simulink model "FBL_commonP_circle"  (R2025a)
settings: Solver=VariableStepAuto  StartTime=0.0  StopTime=240  RelTol=1e-3
undefined symbols (not defined in the file or in its folder): National_Instruments, PCI
libraries: sldrtlib x3, simulink x1
settings Model: Creator=dperera  LastModifiedBy=dperera

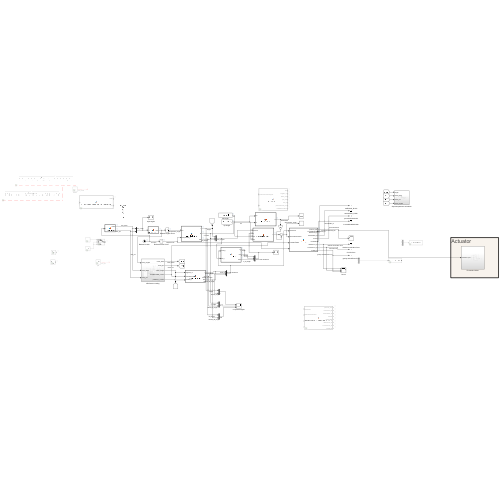
[thumbnail: Simulink's stored preview of the top-level diagram]
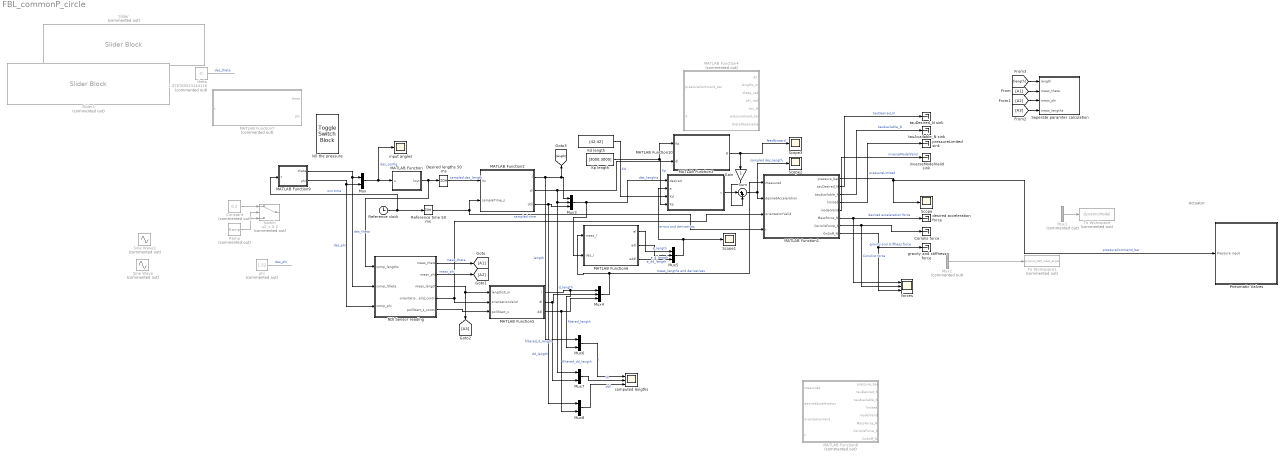
== system FBL_commonP_circle ==
  note: Actuator
  Constant : Constant  Commented=on  Value=0.2
  Coriolis force : Terminator
  Desired lengths 50 ms : ZeroOrderHold  SampleTime=0.05
  Gain : Gain
  Kd length : Constant  Value=[42;42]
  Kp length : Constant  Value=[3000;3000]
  MATLAB Function : MATLAB Function  TreatAsAtomicUnit=on
  MATLAB Function1 : MATLAB Function  TreatAsAtomicUnit=on
  MATLAB Function10 : MATLAB Function  TreatAsAtomicUnit=on
  MATLAB Function2 : MATLAB Function  TreatAsAtomicUnit=on
  MATLAB Function3 : MATLAB Function  TreatAsAtomicUnit=on
  MATLAB Function4 : MATLAB Function  Commented=on  TreatAsAtomicUnit=on
  MATLAB Function5 : MATLAB Function  TreatAsAtomicUnit=on
  MATLAB Function6 : MATLAB Function  TreatAsAtomicUnit=on
  MATLAB Function7 : MATLAB Function  Commented=on  TreatAsAtomicUnit=on
  MATLAB Function8 : MATLAB Function  Commented=on  TreatAsAtomicUnit=on
  MATLAB Function9 : MATLAB Function  TreatAsAtomicUnit=on
  Mux{,6..8} (4 alike) : Mux  Inputs=2
  Mux1 : Mux  Commented=on
  Mux2 : Mux  Commented=on
  Mux3 : Mux  Inputs=3
  Mux4 : Mux  Inputs=3
  Mux5 : Mux  Inputs=3
  NDI Sensor reading : Subsystem
  Pneumatic Valves : Subsystem
  Ramp : simulink/Sources/Ramp  Commented=on  slope=0.2/5  start=1  InitialOutput=0
  Reference clock : Clock
  Reference time 50 ms : ZeroOrderHold  SampleTime=0.05
  Scope{,1..3} (4 alike) : Scope
      Scope settings: ActiveDisplayYMinimum=-0.37334273695648185  ActiveDisplayYMaximum=3.3600846326083369  DataLoggingVariableName=ScopeData6
      Scope1 settings: ActiveDisplayYMinimum=-0.019338012914829127  ActiveDisplayYMaximum=0.016644783463870338  DataLoggingVariableName=ScopeData8
      Scope2 settings: ActiveDisplayYMinimum=-1  ActiveDisplayYMaximum=1  DataLoggingVariableName=ScopeData9
      Scope3 settings: ActiveDisplayYMinimum=-5.4117919345695178  ActiveDisplayYMaximum=5.4108217557534957  DataLoggingVariableName=ScopeData13
  Seperate paramter calculation : Subsystem
  Sine Wave : Sin  Commented=on  Amplitude=1.5  Bias=1.5  Frequency=0.2  Phase=3*pi/2  SampleTime=0
  Sine Wave1 : Sin  Commented=on  Amplitude=1.5  Bias=1.5  Frequency=0.2  Phase=3*pi/2  SampleTime=0
  Slider : SliderBlock  Commented=on  ScaleMin=-3.14  ScaleMax=3.14
  Slider1 : SliderBlock  Commented=on  ScaleMax=3.14
  Sum : Sum  Inputs=|++
  Switch : Switch  Commented=on  Criteria=u2 > Threshold  Threshold=0.2  SaturateOnIntegerOverflow=off  InputSameDT=off
  To Workspace : ToWorkspace  Commented=on  VariableName=dynamicModel  SaveFormat=Timeseries  SampleTime=-1
  To Workspace1 : ToWorkspace  Commented=on  VariableName=dynamic_NDI_meas_angle  SaveFormat=Timeseries  SampleTime=-1
  computed lengths : Scope  NumInputPorts=3
      settings: ActiveDisplayYMinimum=-0.0163263543588523  ActiveDisplayYMaximum=0.016938688313851029  DataLoggingVariableName=ScopeData11
  desired acceleration force : Terminator
  forces : Scope  NumInputPorts=3
      settings: ActiveDisplayYMinimum=-26.920603597626503  ActiveDisplayYMaximum=23.728678964344354  DataLoggingVariableName=ScopeData10
  gravity and stiffness force : Terminator
  input angles : Scope
      settings: ActiveDisplayYMinimum=-0.19634954084936201  ActiveDisplayYMaximum=1.7671458676442586  DataLoggingVariableName=ScopeData12
  inverseModelValid sink : Terminator
  kill the pressure : ToggleSwitchBlock
  phi : Constant  Commented=on  Value=1.52
  pressureLimited sink : Terminator
  tauAvailable_N sink : Terminator
  tauDesired_N sink : Terminator
  theta : Constant  Commented=on  Value=1.076760523144116
  wires:
  Mux/1 -> input angles/1, MATLAB Function/1(u)  "des_config"
  MATLAB Function9/1(theta) -> NDI Sensor reading/2(comp_ltheta), Mux/1  "des_theta"
  Mux1/1 -> To Workspace/1
  Mux2/1 -> To Workspace1/1
  MATLAB Function/1(lout) -> Desired lengths 50 ms/1, NDI Sensor reading/1(comp_lengths)
  NDI Sensor reading/3(meas_length) -> MATLAB Function5/1(lengths3_m), [A3]
  MATLAB Function2/1(l) -> Mux6/1, Mux3/1, [length]  "length"
  MATLAB Function2/2(dl) -> MATLAB Function10/2(dl), Mux7/1, Mux3/2  "d_length"
  MATLAB Function2/3(ddl) -> Mux8/1, Mux3/3  "dd_length"
  MATLAB Function5/1(l) -> Mux6/2, Mux4/1  "fitered_length"
  MATLAB Function5/2(dl) -> Mux7/2, Mux4/2  "filtered_d_length"
  MATLAB Function5/3(ddl) -> Mux8/2, Mux4/3  "filtered_dd_length"
  Mux4/1 -> MATLAB Function1/1(measured), MATLAB Function6/1(meas_l)  "meas_lengths and derivatives"
  Mux3/1 -> MATLAB Function3/1(desired), MATLAB Function6/2(des_l)  "des_lenghts"
  MATLAB Function6/2(edl) -> Mux5/2  "e_d_length"
  MATLAB Function6/1(el) -> Mux5/1  "e_length"
  MATLAB Function6/3(eddl) -> Mux5/3  "e_dd_length"
  Mux5/1 -> MATLAB Function3/2(e), Scope1/1  "errors and derivatives"
  Desired lengths 50 ms/1 -> MATLAB Function2/1(lIn)  "sampled des_length"
  Reference clock/1 -> MATLAB Function9/1(t), Reference time 50 ms/1  "sim time"
  Reference time 50 ms/1 -> MATLAB Function1/4(t), MATLAB Function2/2(sampleTime_s)  "sampled time"
  NDI Sensor reading/4(orientationValid_control) -> MATLAB Function1/3(orientationValid), MATLAB Function5/2(orientationValid)
  NDI Sensor reading/5(pollStart_s_control) -> MATLAB Function5/3(pollStart_s)
  Kd length/1 -> MATLAB Function3/3(Kd)  "Kd"
  Kp length/1 -> MATLAB Function10/1(Kp), MATLAB Function3/4(Kp)  "Kp"
  MATLAB Function3/1(v) -> Sum/1
  MATLAB Function1/1(pressure_bar) -> Scope/1, Pneumatic Valves/1(Pressure input)  "pressureCommand_bar"
  MATLAB Function1/2(tauDesired_N) -> tauDesired_N sink/1  "tauDesired_N"
  MATLAB Function1/3(tauAvailable_N) -> tauAvailable_N sink/1  "tauAvailable_N"
  MATLAB Function1/4(limited) -> pressureLimited sink/1  "pressureLimited"
  MATLAB Function1/5(modelValid) -> inverseModelValid sink/1  "inverseModelValid"
  NDI Sensor reading/1(meas_theta) -> [A1]  "meas_theta"
  [A1] -> Seperate paramter calculation/2(meas_theta)
  NDI Sensor reading/2(meas_phi) -> [A2]  "meas_phi"
  [A2] -> Seperate paramter calculation/3(meas_phi)
  [A3] -> Seperate paramter calculation/4(meas_lengths)
  [length] -> Seperate paramter calculation/1(length)
  MATLAB Function1/6(MassForce_N) -> forces/1, desired acceleration force/1  "desired acceleration force"
  MATLAB Function1/7(CoriolisForce_N) -> forces/2, Coriolis force/1  "Coriolist force"
  MATLAB Function1/8(GnStiff_N) -> forces/3, gravity and stiffness force/1  "gravity and stiffness force"
  Mux6/1 -> computed lengths/1  "l"
  Mux7/1 -> computed lengths/2  "dl"
  Mux8/1 -> computed lengths/3  "ddl"
  Ramp/1 -> Switch/2, Switch/3
  Constant/1 -> Switch/1
  theta/1 -> ?  "des_theta"
  phi/1 -> ?  "des_phi"
  MATLAB Function9/2(phi) -> NDI Sensor reading/3(comp_phi), Mux/2  "des_phi"
  MATLAB Function10/1(ff) -> Scope3/1, Gain/1  "feedforward"
  Sum/1 -> MATLAB Function1/2(desiredAcceleration), Scope2/1  "sampled des_length"
  Gain/1 -> Sum/2

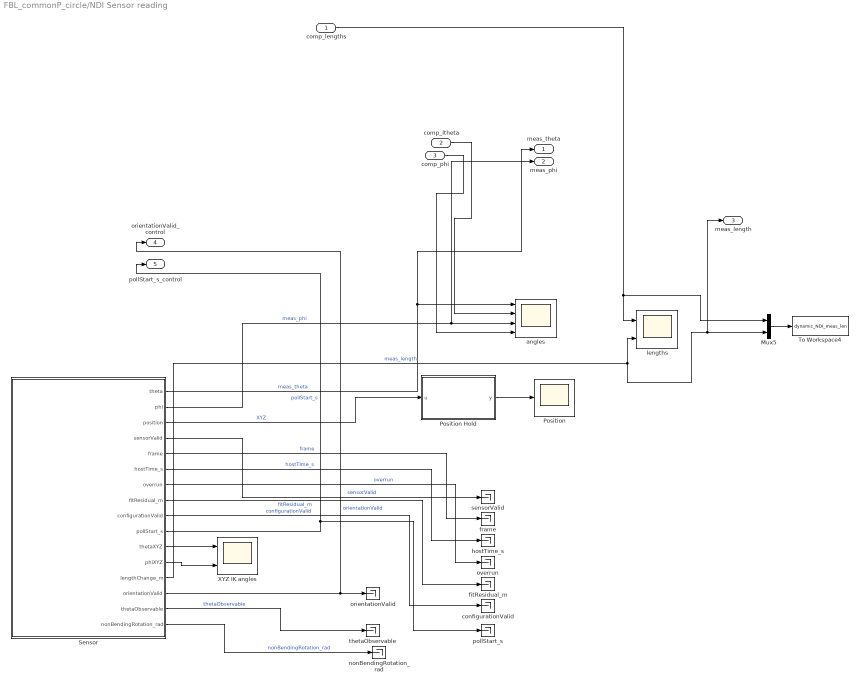
== system FBL_commonP_circle/NDI Sensor reading ==
  comp_lengths : Inport
  comp_ltheta : Inport  Port=2
  comp_phi : Inport  Port=3
  Mux5 : Mux  Inputs=2
  Position : Scope
      settings: ActiveDisplayYMinimum=-0.21656345474719998  ActiveDisplayYMaximum=0.33777835857868188
  Position Hold : MATLAB Function  TreatAsAtomicUnit=on
  Sensor : Subsystem
  To Workspace4 : ToWorkspace  VariableName=dynamic_NDI_meas_len  SaveFormat=Timeseries  SampleTime=-1
  XYZ IK angles : Scope  NumInputPorts=2
      settings: DataLoggingVariableName=ScopeData2
  angles : Scope  NumInputPorts=4
      settings: ActiveDisplayYMinimum=-3.523325206652153  ActiveDisplayYMaximum=4.312344616749975
  configurationValid : Terminator
  fitResidual_m : Terminator
  frame : Terminator
  hostTime_s : Terminator
  lengths : Scope  NumInputPorts=2
      settings: ActiveDisplayYMinimum=-0.0017146774565175815  ActiveDisplayYMaximum=0.0020057370608089205  DataLoggingVariableName=ScopeData3
  nonBendingRotation_rad : Terminator
  orientationValid : Terminator
  overrun : Terminator
  pollStart_s : Terminator
  sensorValid : Terminator
  thetaObservable : Terminator
  meas_theta : Outport
  meas_phi : Outport  Port=2
  meas_length : Outport  Port=3
  orientationValid_control : Outport  Port=4
  pollStart_s_control : Outport  Port=5
  wires:
  Sensor/13(lengthChange_m) -> lengths/2, meas_length/1, Mux5/2  "meas_length"
  comp_lengths/1 -> lengths/1, Mux5/1
  Sensor/10(pollStart_s) -> pollStart_s/1, pollStart_s_control/1  "pollStart_s"
  Sensor/2(phi) -> angles/3, meas_phi/1  "meas_phi"
  Sensor/3(position) -> Position Hold/1(u)  "XYZ"
  Sensor/1(theta) -> meas_theta/1, angles/1  "meas_theta"
  Sensor/6(hostTime_s) -> hostTime_s/1  "hostTIme_s"
  Sensor/9(configurationValid) -> configurationValid/1  "configurationValid"
  Sensor/4(sensorValid) -> sensorValid/1  "sensorValid"
  Sensor/7(overrun) -> overrun/1  "overrun"
  Sensor/5(frame) -> frame/1  "frame"
  comp_ltheta/1 -> angles/2
  Sensor/8(fitResidual_m) -> fitResidual_m/1  "fitResidual_m"
  Sensor/12(phiXYZ) -> XYZ IK angles/2
  Sensor/11(thetaXYZ) -> XYZ IK angles/1
  Position Hold/1(y) -> Position/1
  Mux5/1 -> To Workspace4/1
  Sensor/14(orientationValid) -> orientationValid_control/1, orientationValid/1  "orientationValid"
  Sensor/16(nonBendingRotation_rad) -> nonBendingRotation_rad/1  "nonBendingRotation_rad"
  Sensor/15(thetaObservable) -> thetaObservable/1  "thetaObservable"
  comp_phi/1 -> angles/4

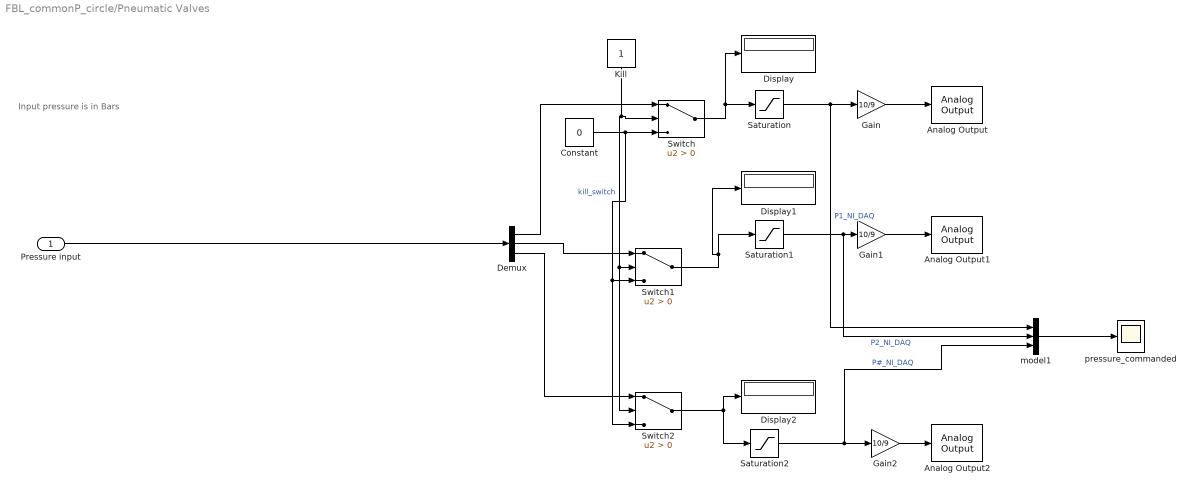
== system FBL_commonP_circle/Pneumatic Valves ==
  note: Input pressure is in Bars
  Pressure input : Inport
  Analog Output : sldrtlib/Analog Output  SampleTime=1/100  MaxMissedTicks=inf  ShowMissedTicks=off  YieldWhenWaiting=off  DrvName=National_Instruments/PCI-6703  DrvAddress=4294967295  DrvOptions=0  Channels=1  RangeMode=1  VoltRange=1  InitialValue=0  FinalValue=0
      settings: AttributesFormatString=National Instruments\nPCI-6703 [auto]
  Analog Output1 : sldrtlib/Analog Output  SampleTime=1/100  MaxMissedTicks=inf  ShowMissedTicks=off  YieldWhenWaiting=off  DrvName=National_Instruments/PCI-6703  DrvAddress=4294967295  DrvOptions=0  Channels=2  RangeMode=1  VoltRange=1  InitialValue=0  FinalValue=0
      settings: AttributesFormatString=National Instruments\nPCI-6703 [auto]
  Analog Output2 : sldrtlib/Analog Output  SampleTime=1/100  MaxMissedTicks=inf  ShowMissedTicks=off  YieldWhenWaiting=off  DrvName=National_Instruments/PCI-6703  DrvAddress=4294967295  DrvOptions=0  Channels=3  RangeMode=1  VoltRange=1  InitialValue=0  FinalValue=0
      settings: AttributesFormatString=National Instruments\nPCI-6703 [auto]
  Constant : Constant  Value=0
  Demux : Demux  Outputs=3
  Display : Display
  Display1 : Display
  Display2 : Display
  Gain : Gain  Gain=10/9
  Gain1 : Gain  Gain=10/9
  Gain2 : Gain  Gain=10/9
  Kill : Constant
  Saturation : Saturate  UpperLimit=3  LowerLimit=0
  Saturation1 : Saturate  UpperLimit=3  LowerLimit=0
  Saturation2 : Saturate  UpperLimit=3  LowerLimit=0
  Switch : Switch  Criteria=u2 > Threshold  SaturateOnIntegerOverflow=off  InputSameDT=off
  Switch1 : Switch  Criteria=u2 > Threshold  SaturateOnIntegerOverflow=off  InputSameDT=off
  Switch2 : Switch  Criteria=u2 > Threshold  SaturateOnIntegerOverflow=off  InputSameDT=off
  model1 : Mux  Inputs=3
  pressure_commanded : Scope
      settings: ActiveDisplayYMinimum=-0.37499999999999989  ActiveDisplayYMaximum=3.375  DataLoggingVariableName=ScopeData7
  wires:
  Constant/1 -> Switch2/3, Switch1/3, Switch/3
  Kill/1 -> Switch2/2, Switch1/2, Switch/2  "kill_switch"
  Switch/1 -> Display/1, Saturation/1
  Gain/1 -> Analog Output/1
  Saturation/1 -> model1/1, Gain/1  "P1_NI_DAQ"
  Demux/3 -> Switch2/1
  Gain1/1 -> Analog Output1/1
  Gain2/1 -> Analog Output2/1
  Saturation2/1 -> model1/3, Gain2/1  "P#_NI_DAQ"
  Switch2/1 -> Saturation2/1, Display2/1
  Demux/2 -> Switch1/1
  Switch1/1 -> Saturation1/1, Display1/1
  model1/1 -> pressure_commanded/1
  Saturation1/1 -> model1/2, Gain1/1  "P2_NI_DAQ"
  Demux/1 -> Switch/1
  Pressure input/1 -> Demux/1

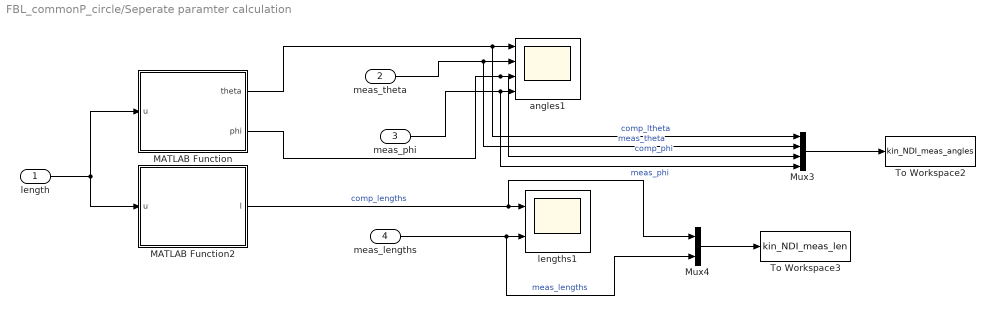
== system FBL_commonP_circle/Seperate paramter calculation ==
  length : Inport
  meas_theta : Inport  Port=2
  meas_phi : Inport  Port=3
  meas_lengths : Inport  Port=4
  MATLAB Function : MATLAB Function  TreatAsAtomicUnit=on
  MATLAB Function2 : MATLAB Function  TreatAsAtomicUnit=on
  Mux3 : Mux
  Mux4 : Mux  Inputs=2
  To Workspace2 : ToWorkspace  VariableName=kin_NDI_meas_angles  SaveFormat=Timeseries  SampleTime=-1
  To Workspace3 : ToWorkspace  VariableName=kin_NDI_meas_len  SaveFormat=Timeseries  SampleTime=-1
  angles1 : Scope  NumInputPorts=4
      settings: ActiveDisplayYMinimum=-3.9269137322662839  ActiveDisplayYMaximum=3.9265599408279468  DataLoggingVariableName=ScopeData4
  lengths1 : Scope  NumInputPorts=2
      settings: ActiveDisplayYMinimum=-0.02243223759551808  ActiveDisplayYMaximum=0.037530111947788623  DataLoggingVariableName=ScopeData5
  wires:
  meas_lengths/1 -> Mux4/2, lengths1/2  "meas_lengths"
  meas_theta/1 -> Mux3/2, angles1/2  "meas_theta"
  MATLAB Function/2(phi) -> Mux3/3, angles1/3  "comp_phi"
  Mux3/1 -> To Workspace2/1
  meas_phi/1 -> Mux3/4, angles1/4  "meas_phi"
  MATLAB Function/1(theta) -> Mux3/1, angles1/1  "comp_ltheta"
  Mux4/1 -> To Workspace3/1
  MATLAB Function2/1(l) -> Mux4/1, lengths1/1  "comp_lengths"
  length/1 -> MATLAB Function2/1(u), MATLAB Function/1(u)

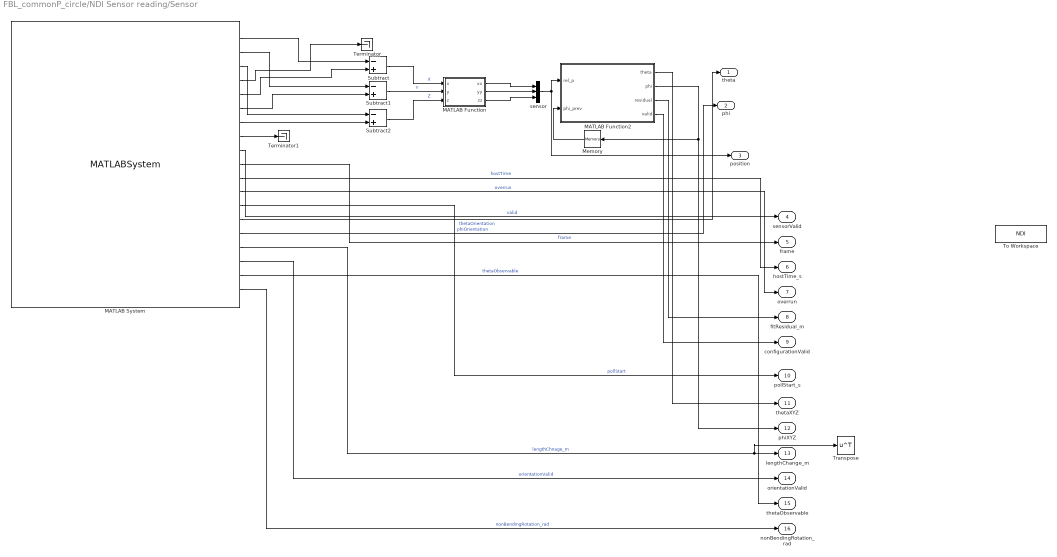
== system FBL_commonP_circle/NDI Sensor reading/Sensor ==
  MATLAB Function : MATLAB Function  TreatAsAtomicUnit=on
  MATLAB Function2 : MATLAB Function  TreatAsAtomicUnit=on
  MATLAB System : MATLABSystem  System=AuroraReader_s2_Position_only  Port=COM12  BaudRate=ndiConfig.BaudRate  SamplePeriod=ndiConfig.SamplePeriod  BaseSensorId=0A  TipSensorId=0B  CalibrationFile=C:\Users\dperera\OneDrive - Texas A&M University\Lab\Research\fDyn_ExpCom\hyDyn_Ctrl\ndi_orientation_recordings\calibration_20260930_190505_898.mat  PreflightSeconds=5  ActuatorRadius=0.013  SimulateUsing=Interpreted execution
      mask Type: AuroraReader_s2_Position_only
  Memory : Memory  InitialCondition=0.0001
  Subtract : Sum  Inputs=-+
  Subtract1 : Sum  Inputs=-+
  Subtract2 : Sum  Inputs=-+
  Terminator : Terminator
  Terminator1 : Terminator
  To Workspace : ToWorkspace  VariableName=NDI  SaveFormat=Timeseries  SampleTime=-1
  Transpose : Math  Operator=transpose
  sensor : Mux  Inputs=3
  theta : Outport
  phi : Outport  Port=2
  position : Outport  Port=3
  sensorValid : Outport  Port=4
  frame : Outport  Port=5
  hostTime_s : Outport  Port=6
  overrun : Outport  Port=7
  fitResidual_m : Outport  Port=8
  configurationValid : Outport  Port=9
  pollStart_s : Outport  Port=10
  thetaXYZ : Outport  Port=11
  phiXYZ : Outport  Port=12
  lengthChange_m : Outport  Port=13
  orientationValid : Outport  Port=14
  thetaObservable : Outport  Port=15
  nonBendingRotation_rad : Outport  Port=16
  wires:
  MATLAB System/2 -> Subtract1/1
  MATLAB Function/3(zz) -> sensor/3
  Subtract1/1 -> MATLAB Function/2(y)  "Y"
  Subtract2/1 -> MATLAB Function/3(z)  "Z"
  MATLAB System/5 -> Subtract/2
  sensor/1 -> position/1, MATLAB Function2/1(rel_p)
  MATLAB System/8 -> Terminator1/1
  MATLAB Function/1(xx) -> sensor/1
  Subtract/1 -> MATLAB Function/1(x)  "X"
  MATLAB Function/2(yy) -> sensor/2
  MATLAB System/1 -> Subtract/1
  MATLAB Function2/2(phi) -> Memory/1, phiXYZ/1
  MATLAB System/7 -> Subtract2/2
  MATLAB System/4 -> Terminator/1
  MATLAB System/3 -> Subtract2/1
  MATLAB System/6 -> Subtract1/2
  Memory/1 -> MATLAB Function2/2(phi_prev)
  MATLAB System/9 -> sensorValid/1  "valid"
  MATLAB System/11 -> hostTime_s/1  "hostTime"
  MATLAB System/12 -> overrun/1  "overrun"
  MATLAB Function2/3(residual) -> fitResidual_m/1
  MATLAB Function2/4(valid) -> configurationValid/1
  MATLAB System/13 -> pollStart_s/1  "pollStart"
  MATLAB System/14 -> theta/1  "thetaOrientation"
  MATLAB System/15 -> phi/1  "phiOrientation"
  MATLAB Function2/1(theta) -> thetaXYZ/1
  MATLAB System/16 -> Transpose/1, lengthChange_m/1  "lengthChnage_m"
  MATLAB System/17 -> orientationValid/1  "orientationValid"
  MATLAB System/18 -> thetaObservable/1  "thetaObservable"
  MATLAB System/19 -> nonBendingRotation_rad/1  "nonBendingRotation_rad"
  MATLAB System/10 -> frame/1  "frame"

== matlab function FBL_commonP_circle/MATLAB Function2 ==
  data: lIn input; l output; dl output; ddl output; sampleTime_s input
function [l, dl, ddl] = lengthDerivatives(lIn, sampleTime_s)
%#codegen
% Desired reduced lengths [l2;l3] in m; derivatives in m/s and m/s^2.
% sampleTime_s is a 0.05 s zero-order-held Clock signal.
persistent lastL lastT velocity acceleration
if isempty(lastT)
    lastL = zeros(2,1);
    lastT = -1;
    velocity = zeros(2,1);
    acceleration = zeros(2,1);
end
l = lastL;
dl = velocity;
ddl = acceleration;
if ~all(isfinite(lIn)) || ~isfinite(sampleTime_s)
    return;
end
q = [lIn(1); lIn(2)];
if lastT < 0
    lastL = q;
    lastT = sampleTime_s;
    l = q;
    return;
end
dt = sampleTime_s - lastT;
if dt > 1e-6
    rawVelocity = (q-lastL)/dt;
    oldVelocity = velocity;
    alphaV = dt/(0.10+dt);
    velocity = velocity + alphaV*(rawVelocity-velocity);
    rawAcceleration = (velocity-oldVelocity)/dt;
    alphaA = dt/(0.15+dt);
    acceleration = acceleration + alphaA*(rawAcceleration-acceleration);
    lastL = q;
    lastT = sampleTime_s;
end
l = lastL;
dl = velocity;
ddl = acceleration;
end

== matlab function FBL_commonP_circle/MATLAB Function3 ==
  data: desired input; v output; e input; Kd input; Kp input
function v = feedbacklinearization(desired, e, Kd, Kp)
%#codegen
% v = desired acceleration + Kd*velocity error + Kp*position error.
% desired,e: [l2;l3;dl2;dl3;ddl2;ddl3]; gains are 2-vectors.
% Kd units 1/s, Kp units 1/s^2; v units m/s^2.
v = zeros(2,1);
if ~all(isfinite(desired)) || ~all(isfinite(e)) || ...
        ~all(isfinite(Kd)) || ~all(isfinite(Kp)) || ...
        any(Kd < 0) || any(Kp < 0)
    return;
end
v = desired(5:6) + Kd(:).*e(3:4) + Kp(:).*e(1:2);
end

== matlab function FBL_commonP_circle/MATLAB Function4 ==
  data: pressureCommand_bar input; X input; dX output; lengths_m output; theta_rad output; phi_rad output; tau_N output; pressureUsed_bar output; thetaObservable output
% function dX  = DynamicModel(p, X)
%#codegen
% This file computes length velocity and accelration from pressures using the dynamic model.
%
% Inputs:
%   p   : pressures [3x1] (Pa)
%   X   : length derivatives [4x1] (m)
%         [l2; l3; dl2; dl3]
%
% Output:
%   dX  : length derivatives [4x1] (m)
%         [dl2; dl3; ddl2; ddl3]

function [dX, lengths_m, theta_rad, phi_rad, tau_N, ...
          pressureUsed_bar, thetaObservable] = forwardModel(pressureCommand_bar, X)
%#codegen
% pressureCommand_bar = [P1; P2; P3], nonnegative bar
% X = [l2; l3; dl2; dl3], with l1 = -l2-l3

L = 0.17411;
r = 0.013; % PMA radial offset from backbone (m)
mass = 0.1;
K = 1350 * [2 1; 1 2];
D = 40 * eye(2);
gArm = [0; 0; -9.81];
mu = 2000;
lengthBounds = [-0.035; 0.035; 1e6];

pressureUsed_bar = min(max(pressureCommand_bar, 0), 3);
pressureDiameter_m = 0.013; % Effective pressure-area diameter, independent of r
pressureRadius_m = pressureDiameter_m/2;
area = pi * pressureRadius_m^2;

% Positive P1, P2, P3 give the established -X, -60°, +60°
% nominal bending directions, respectively.
tau_N = area * 1e5 * [-1 1 0; -1 0 1] * pressureUsed_bar;

dX = armS_single_entry(0, X, L, r, mass, gArm, ...
                       K, D, tau_N, mu, lengthBounds);

l2 = X(1);
l3 = X(2);
lengths_m = [-l2-l3; l2; l3];

u = (l2+l3)/r;
v = (l3-l2)/(sqrt(3)*r);
phi_rad = hypot(u, v);
theta_rad = atan2(v, u);
thetaObservable = phi_rad > 0.5*pi/180;


end

== matlab function FBL_commonP_circle/MATLAB Function5 ==
  data: lengths3_m input; l output; dl output; ddl output; orientationValid input; pollStart_s input
function [l, dl, ddl] = filteredDerivatives(lengths3_m, orientationValid, pollStart_s)
%#codegen
% NDI lengths are [l1;l2;l3]; model coordinates are [l2;l3].
% Invalid or repeated BX frames do not update the derivative states.
persistent lastL lastT velocity acceleration
if isempty(lastT)
    lastL = nan(2,1);
    lastT = -1;
    velocity = zeros(2,1);
    acceleration = zeros(2,1);
end
l = lastL;
dl = velocity;
ddl = acceleration;
if ~orientationValid || ~all(isfinite(lengths3_m)) || ~isfinite(pollStart_s)
    return;
end
q = [lengths3_m(2); lengths3_m(3)];
if lastT < 0
    lastL = q;
    lastT = pollStart_s;
    l = q;
    return;
end
dt = pollStart_s-lastT;
if dt > 1e-6
    rawVelocity = (q-lastL)/dt;
    oldVelocity = velocity;
    alphaV = dt/(0.20+dt);
    velocity = velocity + alphaV*(rawVelocity-velocity);
    rawAcceleration = (velocity-oldVelocity)/dt;
    alphaA = dt/(0.30+dt);
    acceleration = acceleration + alphaA*(rawAcceleration-acceleration);
    lastL = q;
    lastT = pollStart_s;
end
l = lastL;
dl = velocity;
ddl = acceleration;
end

== matlab function FBL_commonP_circle/MATLAB Function6 ==
  data: meas_l input; el output; edl output; eddl output; des_l input
function [el, edl, eddl] = computeLengthError(meas_l, des_l)
%#codegen
% Inputs: [l2;l3;dl2;dl3;ddl2;ddl3].
% Subtract the filtered rates directly: differentiation of position error
% would amplify NDI noise and repeat samples.
el = nan(2,1);
edl = nan(2,1);
eddl = nan(2,1);
if ~all(isfinite(meas_l)) || ~all(isfinite(des_l))
    return;
end
el = des_l(1:2)-meas_l(1:2);
edl = des_l(3:4)-meas_l(3:4);
eddl = des_l(5:6)-meas_l(5:6);
end

== matlab function FBL_commonP_circle/MATLAB Function7 ==
  data: t input; theta output; phi output
function [theta, phi] = commonPressureFeedbackReferenceBlock(t)
%#codegen
% Paste into the existing thetaCircle MATLAB Function block in a COPY of
% the feedback-linearization model. Connect theta and phi to the desired
% angle Mux and NDI comparison inputs; bypass the old circle/ramp sources.
% Stop Time: 240 s. Both reference steps are only 0.01 rad.

theta = 0.0;
phi = 0.0;
if ~isfinite(t) || t < 0.0
    return;
end

if t >= 90.0 && t < 130.0
    theta = 0.0; % U-direction bend.
    if t < 95.0
        u = (t-90.0)/5.0;
        phi = 0.01*u*u*(3.0-2.0*u);
    elseif t < 125.0
        phi = 0.01;
    else
        u = (t-125.0)/5.0;
        phi = 0.01*(1.0-u*u*(3.0-2.0*u));
    end
elseif t >= 160.0 && t < 200.0
    theta = pi/2; % V-direction bend.
    if t < 165.0
        u = (t-160.0)/5.0;
        phi = 0.01*u*u*(3.0-2.0*u);
    elseif t < 195.0
        phi = 0.01;
    else
        u = (t-195.0)/5.0;
        phi = 0.01*(1.0-u*u*(3.0-2.0*u));
    end
end
end

== matlab function FBL_commonP_circle/MATLAB Function8 ==
  data: measured input; desiredAcceleration input; pressure_bar output; tauDesired_N output; tauAvailable_N output; limited output; modelValid output; orientationValid input; MassForce_N output; CoriolisForce_N output; GnStiff_N output; t input
function [pressure_bar, tauDesired_N, tauAvailable_N, limited, modelValid, ...
    MassForce_N, CoriolisForce_N, GnStiff_N] = ...
    commonPressureFeedbackInverseBlock(measured, desiredAcceleration, orientationValid, t)
%#codegen
% Paste into the existing inverseModel MATLAB Function block in a COPY of
% the feedback-linearization model. Add Clock time t as the fourth input.
% Outputs and their order match the existing block.
%
% Test sequence: zero 0-10 s, fixed trial-4 trim 10-50 s, bounded
% feedback 50-220 s, zero after 220 s. Set model Stop Time to 240 s.
% The block rate-limits each pressure command to +/-0.8 bar/s.

pressure_bar = zeros(3,1);
tauDesired_N = zeros(2,1);
tauAvailable_N = zeros(2,1);
MassForce_N = zeros(2,1);
CoriolisForce_N = zeros(2,1);
GnStiff_N = zeros(2,1);
limited = false;
modelValid = false;

persistent tauAnchor_N anchorReady lastPressure_bar lastTime_s
if isempty(anchorReady)
    tauAnchor_N = zeros(2,1);
    anchorReady = false;
    lastPressure_bar = zeros(3,1);
    lastTime_s = -1.0;
end

if ~isfinite(t) || t < 0.0 || ...
        ~orientationValid || ~all(isfinite(measured(1:4))) || ...
        ~all(isfinite(desiredAcceleration))
    % Keep the model's fail-to-zero behavior on invalid NDI/model input.
    lastPressure_bar = zeros(3,1);
    if isfinite(t), lastTime_s = t; end
    return;
end

q = measured(1:2);
dq = measured(3:4);
params.N = 1;
params.L = 0.17411;
params.r = 0.013; % Radial PMA offset, not pressure-area radius.
params.mi = 0.1;
params.g = [0;0;-9.81];
params.K = 650*[2 1;1 2];
params.D = 40*eye(2);
params.mu = 2000;
params.lKbounds = [-0.035;0.035;1e6];
[M,C,G] = armS_single_core(q,dq,params);
Keff = params.K;
for i = 1:2
    Keff(i,i) = Keff(i,i) + 0.5*params.lKbounds(3)*(2 + ...
        tanh(params.mu*(q(i)-params.lKbounds(2))) - ...
        tanh(params.mu*(q(i)-params.lKbounds(1))));
end

MassForce_N = M*desiredAcceleration;
CoriolisForce_N = (C+params.D)*dq;
GnStiff_N = G+Keff*q;
tauDesired_N = MassForce_N+CoriolisForce_N+GnStiff_N;
if ~all(isfinite(tauDesired_N)) || ~all(isfinite(GnStiff_N))
    tauDesired_N = zeros(2,1);
    lastPressure_bar = zeros(3,1);
    lastTime_s = t;
    return;
end
modelValid = true;

common_bar = 1.6;
s0_bar = -0.0983981693363845;
a0_bar = -0.0819816714043049;
maxDeltaS_bar = 0.04;
maxDeltaA_bar = 0.04;
pressureRate_barPerS = 0.8;
forcePerBar_N = pi*(0.013/2)^2*1e5;

target_bar = zeros(3,1);
if t >= 10.0 && t < 220.0
    ds_bar = 0.0;
    da_bar = 0.0;
    if t >= 50.0
        if ~anchorReady
            % Anchor only the nominal static model force at the settled
            % trim. Do not cancel the PD correction to the desired pose.
            tauAnchor_N = GnStiff_N;
            anchorReady = true;
        end
        deltaTau_N = tauDesired_N-tauAnchor_N;
        dsWanted_bar = (deltaTau_N(1)+deltaTau_N(2))/(2*forcePerBar_N);
        daWanted_bar = (deltaTau_N(2)-deltaTau_N(1))/(2*forcePerBar_N);
        ds_bar = min(max(dsWanted_bar,-maxDeltaS_bar),maxDeltaS_bar);
        da_bar = min(max(daWanted_bar,-maxDeltaA_bar),maxDeltaA_bar);
        limited = abs(ds_bar-dsWanted_bar)>1e-12 || ...
            abs(da_bar-daWanted_bar)>1e-12;
        % Gradually engage feedback after the static trim hold.
        u = min(max((t-50.0)/5.0,0.0),1.0);
        blend = u*u*(3.0-2.0*u);
        ds_bar = blend*ds_bar;
        da_bar = blend*da_bar;
    end
    s_bar = s0_bar+ds_bar;
    a_bar = a0_bar+da_bar;
    target_bar = [common_bar-(2.0/3.0)*s_bar; ...
                  common_bar+(1.0/3.0)*s_bar-a_bar; ...
                  common_bar+(1.0/3.0)*s_bar+a_bar];
    bounded = min(max(target_bar,1.2),3.0);
    if any(abs(bounded-target_bar)>1e-12), limited = true; end
    target_bar = bounded;
end

% Discrete state implements a per-channel slew limit using Clock time.
% The initial trim takes about 2.1 s to reach its target.
if lastTime_s < 0.0 || t < lastTime_s
    lastPressure_bar = zeros(3,1);
    lastTime_s = t;
end
dt = t-lastTime_s;
if dt > 0.0
    step_bar = pressureRate_barPerS*dt;
    pressure_bar = min(max(target_bar, ...
        lastPressure_bar-step_bar),lastPressure_bar+step_bar);
    lastPressure_bar = pressure_bar;
    lastTime_s = t;
else
    pressure_bar = lastPressure_bar;
end
if any(abs(pressure_bar-target_bar)>1e-9), limited = true; end

% All three active channels have the same nominal 0.8 bar deadzone, so
% their pressure differences give the ideal generalized force directly.
tauAvailable_N = forcePerBar_N * ...
    [pressure_bar(2)-pressure_bar(1); ...
     pressure_bar(3)-pressure_bar(1)];
end

== matlab function FBL_commonP_circle/MATLAB Function9 ==
  data: t input; theta output; phi output
function [theta, phi] = thetaCircle(t)
%#codegen

% Edit these values before each run
des_phi = 1.0;          % rad
circle_time_s = 10.0;   % seconds per circle
num_circles = 5;        % positive integer

theta = 0.0;
phi = 0.0;

if ~isfinite(t) || t < 0.0
    return;
end

circle_start = 10.0;
circle_end = circle_start + num_circles*circle_time_s;
phi_end = circle_end + 20.0;

if t < 5.0
    return;
elseif t < 10.0
    u = (t - 5.0)/5.0;
    phi = des_phi*u*u*(3.0 - 2.0*u);
elseif t < circle_start
    phi = des_phi;
elseif t < circle_end
    progress = (t - circle_start)/circle_time_s;
    lap = floor(progress);
    u = progress - lap;

    theta = 2*pi*(lap + u*u*(3.0 - 2.0*u));
    phi = des_phi;
elseif t < phi_end
    u = (t - circle_end)/20.0;
    theta = 2*pi*num_circles;
    phi = des_phi*(1.0 - u*u*(3.0 - 2.0*u));
end
end

== matlab function FBL_commonP_circle/MATLAB Function10 ==
  data: Kp input; dl input; ff output
function ff = Feedforward(Kp, dl)
%#codegen
ff = zeros(2,1);
if ~all(isfinite(dl)) || ~all(isfinite(Kp)) || any(Kp < 0)
    return;
end
dl = dl(:);
ff =  Kp(:).*dl*0.12;
end

== matlab function FBL_commonP_circle/MATLAB Function1 ==
  data: measured input; desiredAcceleration input; orientationValid input; t input; pressure_bar output; tauDesired_N output; tauAvailable_N output; limited output; modelValid output; MassForce_N output; CoriolisForce_N output; GnStiff_N output
function [pressure_bar, tauDesired_N, tauAvailable_N, limited, modelValid, ...
    MassForce_N, CoriolisForce_N, GnStiff_N] = ...
    commonPressureFeedbackInverseBlockV2(measured, desiredAcceleration, orientationValid, t)
%#codegen
% Paste this entire function into the existing inverseModel MATLAB Function
% block. Inputs and all eight outputs retain the V1 order. Keep the current
% 0.01 rad reference block and the external physical Kill path unchanged.
%
% Test sequence: zero 0-10 s, fixed trial-4 trim 10-50 s, bounded
% feedback 50-220 s, zero after 220 s. Set model Stop Time to 240 s.
% One missing 0.05 s NDI frame holds the previous command. If valid model
% data does not return within 0.10 s of the last valid sample, the fault
% latches and pressure slews to zero at 0.8 bar/s. Restart the simulation
% to clear a latched fault; the separate Kill path remains available.

pressure_bar = zeros(3,1);
tauDesired_N = zeros(2,1);
tauAvailable_N = zeros(2,1);
MassForce_N = zeros(2,1);
CoriolisForce_N = zeros(2,1);
GnStiff_N = zeros(2,1);
limited = false;
modelValid = false;

persistent tauAnchor_N anchorReady lastPressure_bar lastTime_s ...
    lastGoodTime_s faultLatched
if isempty(anchorReady)
    tauAnchor_N = zeros(2,1);
    anchorReady = false;
    lastPressure_bar = zeros(3,1);
    lastTime_s = -1.0;
    lastGoodTime_s = -1.0;
    faultLatched = false;
end

if ~isfinite(t) || t < 0.0
    % Without a usable Clock value a time-based slew cannot be calculated.
    % This exceptional path commands zero; the external Kill remains primary.
    lastPressure_bar = zeros(3,1);
    lastTime_s = -1.0;
    faultLatched = true;
    return;
end

if lastTime_s >= 0.0 && t < lastTime_s
    % A new simulation run starts a new pressure/fault state.
    tauAnchor_N = zeros(2,1);
    anchorReady = false;
    lastPressure_bar = zeros(3,1);
    lastTime_s = -1.0;
    lastGoodTime_s = -1.0;
    faultLatched = false;
end

inputValid = orientationValid && all(isfinite(measured(1:4))) && ...
    all(isfinite(desiredAcceleration));
if inputValid && ~faultLatched
    q = measured(1:2);
    dq = measured(3:4);
    params.N = 1;
    params.L = 0.17411;
    params.r = 0.013; % Radial PMA offset, not pressure-area radius.
    params.mi = 0.1;
    params.g = [0;0;-9.81];
    params.K = 650*[2 1;1 2];
    params.D = 40*eye(2);
    params.mu = 2000;
    params.lKbounds = [-0.035;0.035;1e6];
    [M,C,G] = armS_single_core(q,dq,params);
    Keff = params.K;
    for i = 1:2
        Keff(i,i) = Keff(i,i) + 0.5*params.lKbounds(3)*(2 + ...
            tanh(params.mu*(q(i)-params.lKbounds(2))) - ...
            tanh(params.mu*(q(i)-params.lKbounds(1))));
    end

    MassForce_N = M*desiredAcceleration;
    CoriolisForce_N = (C+params.D)*dq;
    GnStiff_N = G+Keff*q;
    tauDesired_N = MassForce_N+CoriolisForce_N+GnStiff_N;
    modelValid = all(isfinite(tauDesired_N)) && ...
        all(isfinite(GnStiff_N)) && all(isfinite(MassForce_N)) && ...
        all(isfinite(CoriolisForce_N));
    if ~modelValid
        tauDesired_N = zeros(2,1);
        MassForce_N = zeros(2,1);
        CoriolisForce_N = zeros(2,1);
        GnStiff_N = zeros(2,1);
    else
        lastGoodTime_s = t;
    end
end

common_bar = 1.6;
s0_bar = -0.0983981693363845;
a0_bar = -0.0819816714043049;
maxDeltaS_bar = 2.5;
maxDeltaA_bar = 2.5;
pressureRate_barPerS = 2;
forcePerBar_N = pi*(0.013/2)^2*1e5;

target_bar = zeros(3,1);
if ~modelValid
    if ~faultLatched && lastGoodTime_s >= 0.0 && ...
            t-lastGoodTime_s <= 0.10+1e-9
        % A brief invalid frame cannot change the command or anchor.
        target_bar = lastPressure_bar;
    else
        % Sustained invalid data stays faulted until simulation restart.
        faultLatched = true;
    end
elseif ~faultLatched && t < 220.0
    ds_bar = 0.0;
    da_bar = 0.0;
    if t >= 0.0
        if ~anchorReady
            % Anchor only the nominal static model force at the settled
            % trim. Do not cancel the PD correction to the desired pose.
            tauAnchor_N = GnStiff_N;
            anchorReady = true;
        end
        deltaTau_N = tauDesired_N-tauAnchor_N;
        dsWanted_bar = (deltaTau_N(1)+deltaTau_N(2))/(2*forcePerBar_N);
        daWanted_bar = (deltaTau_N(2)-deltaTau_N(1))/(2*forcePerBar_N);
        ds_bar = min(max(dsWanted_bar,-maxDeltaS_bar),maxDeltaS_bar);
        da_bar = min(max(daWanted_bar,-maxDeltaA_bar),maxDeltaA_bar);
        limited = abs(ds_bar-dsWanted_bar)>1e-12 || ...
            abs(da_bar-daWanted_bar)>1e-12;
        % Gradually engage feedback after the static trim hold.
        u = min(max(t/5.0,0.0),1.0);
        blend = u*u*(3.0-2.0*u);
        ds_bar = blend*ds_bar;
        da_bar = blend*da_bar;
    end
    s_bar = s0_bar+ds_bar;
    a_bar = a0_bar+da_bar;
    target_bar = [common_bar-(2.0/3.0)*s_bar; ...
                  common_bar+(1.0/3.0)*s_bar-a_bar; ...
                  common_bar+(1.0/3.0)*s_bar+a_bar];
    bounded = min(max(target_bar,0.2),3.0);
    if any(abs(bounded-target_bar)>1e-12), limited = true; end
    target_bar = bounded;
end

% Discrete state implements a per-channel slew limit using Clock time.
% The initial trim takes about 2.1 s to reach its target.
if lastTime_s < 0.0 || t < lastTime_s
    lastPressure_bar = zeros(3,1);
    lastTime_s = t;
end
dt = t-lastTime_s;
if dt > 0.0
    step_bar = pressureRate_barPerS*dt;
    pressure_bar = min(max(target_bar, ...
        lastPressure_bar-step_bar),lastPressure_bar+step_bar);
    lastPressure_bar = pressure_bar;
    lastTime_s = t;
else
    pressure_bar = lastPressure_bar;
end
if any(abs(pressure_bar-target_bar)>1e-9), limited = true; end

% All three active channels have the same nominal 0.8 bar deadzone, so
% their pressure differences give the ideal generalized force directly.
tauAvailable_N = forcePerBar_N * ...
    [pressure_bar(2)-pressure_bar(1); ...
     pressure_bar(3)-pressure_bar(1)];
end

== matlab function FBL_commonP_circle/Seperate paramter calculation/MATLAB Function ==
  data: u input; theta output; phi output
function [theta, phi] = length2config(u)
%#codegen
% This file convert the length changes into theta/phi
%
% Inputs:
%   u       : length change[2x1] (m)
%             [l2; l3]
%
% Outputs:
%   theta   : bending direction [constant] (rad)
%   phi     : bending amount [constant] (rad)

l = [0.0; u(1); u(2)];
r  = 0.013;

c = [atan2(l(3) - l(2), sqrt(0.3e1) * (l(2) + l(3)));
    0.2e1 / 0.3e1 / r * sqrt((3 * l(2) ^ 2 + 3 * l(3) * l(2) + 3 * l(3) ^ 2))];

theta = c(1);
phi = c(2);

end

== matlab function FBL_commonP_circle/Seperate paramter calculation/MATLAB Function2 ==
  data: u input; l output
function l = lengthVector(u)
%#codegen
% This file create the length vector
%
% Inputs:
%   u       : length change[2x1] (m)
%             [l2; l3]
%
% Outputs:
%   l   : bending direction [3x1] (m)

l = [-(u(1) + u(2)); u(1); u(2)];

end

== matlab function FBL_commonP_circle/NDI Sensor reading/Position Hold ==
  data: u input; y output
function y = fcn(u)
persistent lastPosition
if isempty(lastPosition), lastPosition=nan(3,1); end
if all(isfinite(u)), lastPosition=u; end
y=lastPosition;
end

== matlab function FBL_commonP_circle/NDI Sensor reading/Sensor/MATLAB Function ==
  data: x input; xx output; y input; z input; yy output; zz output
function [xx,yy,zz] = rotateX90(x,y,z)

    R = [1 0 0;
         0 0 1;
         0 -1 0];

    p = R*[x;y;z]*0.001;

    xx=p(1);
    yy=p(2);
    zz=p(3);

    
end

== matlab function FBL_commonP_circle/NDI Sensor reading/Sensor/MATLAB Function2 ==
  data: rel_p input; theta output; phi output; phi_prev input; residual output; valid output
function [theta,phi,residual,valid] = xyz2ThetaPhi(rel_p,phi_prev)
persistent lastPhi lastTheta lastOutputTheta lastOutputPhi lastResidual
if isempty(lastPhi)
    lastPhi=0.0001; lastTheta=0;
    lastOutputTheta=NaN; lastOutputPhi=NaN; lastResidual=NaN;
end
% Keep the external memory for compatibility; never use its NaN.
if isfinite(phi_prev), lastPhi=phi_prev; end
[theta,phi,residual,valid]=ndiSupportFnc.configuration(rel_p,lastPhi,lastTheta);
if valid
    lastPhi=phi; lastTheta=theta;
    lastOutputTheta=theta; lastOutputPhi=phi; lastResidual=residual;
else
    % Scope outputs hold, but configurationValid remains false.
    theta=lastOutputTheta; phi=lastOutputPhi; residual=lastResidual;
end
end

== matlab function FBL_commonP_circle/MATLAB Function ==
  data: u input; lout output
function lout = config2length(u)
%#codegen
% Convert configuration variables to length changes
% Input (u):
%   u       : theta and phi [2x1] (rad)
%               theta angle (rad) [constant]
%               phi angle (rad) [constant]
%   r       : radial offset (m) [constant]
% 
% Output:
%   lout    : lenght changes (m) [s,1]


theta = u(1);
phi = u(2);
r = 0.013;

l = [-r * cos(theta) * phi;
    (0.5e0 * r * cos(theta) - sqrt(0.3e1) * r * sin(theta) / 0.2e1) * phi;
    (0.5e0 * r * cos(theta) + sqrt(0.3e1) * r * sin(theta) / 0.2e1) * phi];

lout = [l(2); l(3)];

end
